simulink model "anjaneya_V5_2026-08-11"  (R2025a)
settings: Solver=VariableStepAuto  StartTime=0.0  StopTime=100  MaxStep=1e-3  RelTol=1e-6
settings Model: Creator=kuppa  LastModifiedBy=kuppa

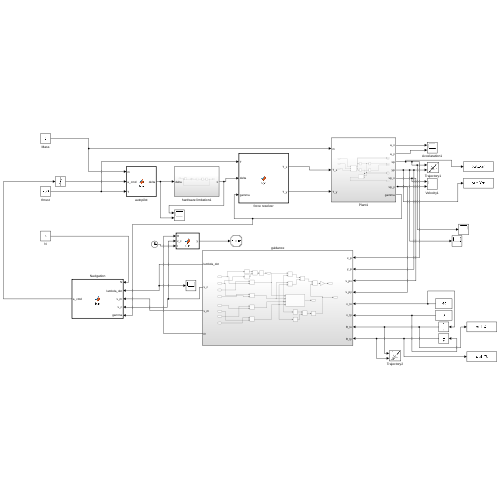
[thumbnail: Simulink's stored preview of the top-level diagram]
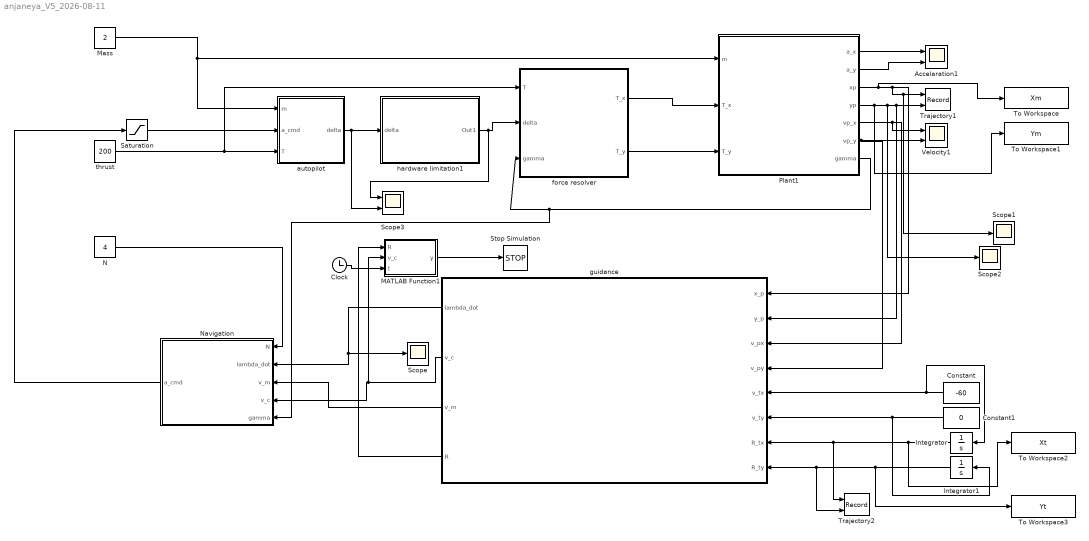
== system anjaneya_V5_2026-08-11 ==
  Accelaration1 : Scope  NumInputPorts=2
      settings: ActiveDisplayYMinimum=-670.09529615601855  ActiveDisplayYMaximum=430.47468331187889  DataLoggingVariableName=ScopeData2
  Clock : Clock
  Constant : Constant  Value=-60
  Constant1 : Constant  Value=0
  Integrator : Integrator  InitialCondition=3000
  Integrator1 : Integrator  InitialCondition=1500
  MATLAB Function1 : MATLAB Function  TreatAsAtomicUnit=on
  Mass : Constant  Value=2
  N : Constant  Value=4
  Navigation : MATLAB Function  TreatAsAtomicUnit=on
  Plant1 : Subsystem
  Saturation : Saturate  UpperLimit=108  LowerLimit=-108
  Scope : Scope
      settings: ActiveDisplayYMinimum=-0.71496170094090172  ActiveDisplayYMaximum=0.65598998004867615
  Scope1 : Scope
      settings: ActiveDisplayYMinimum=-25.430213641107127  ActiveDisplayYMaximum=35.257283778105105
  Scope2 : Scope
      settings: ActiveDisplayYMinimum=-57949.429144793568  ActiveDisplayYMaximum=306802.48338816618  DataLoggingVariableName=ScopeData4
  Scope3 : Scope  NumInputPorts=2
      settings: ActiveDisplayYMinimum=-0.11805254767904227  ActiveDisplayYMaximum=1.5944941621160178  DataLoggingVariableName=ScopeData5
  Stop Simulation : Stop
  To Workspace : ToWorkspace  VariableName=Xm  SaveFormat=Timeseries  SampleTime=-1
  To Workspace1 : ToWorkspace  VariableName=Ym  SaveFormat=Timeseries  SampleTime=-1
  To Workspace2 : ToWorkspace  VariableName=Xt  SaveFormat=Timeseries  SampleTime=-1
  To Workspace3 : ToWorkspace  VariableName=Yt  SaveFormat=Timeseries  SampleTime=-1
  Trajectory1 : Record  NumPorts=2.0  FileSettingsInternal="{\"entries\":[{\"content\":{\"excelSettings\":{\"content\":{},\"type\":\"Streamout.ExcelSettings\"},\"parquetSettings\":{\"content\":{},\"type\":\"Streamout.ParquetSettings\"}},\"type\":\"Streamout.FileSettingStorage\",\"uuid\":\"\"}],\"packageUris\":[\"http:\\/\\/schema.mathworks.com\\/mf0\\/streamout_blocks\\/R2020a\"],\"version\":\"1.0\"}"  FrameSettings=[0, 0]  Layout=[1 1]  SignalsInternal="{\"entries\":[{\"content\":{\"signals\":[{\"content\":{\"blockPath\":[],\"dimensions\":[1],\"domain\":\"\",\"lineColor\":\"#0072bd\",\"lineWidth\":2,\"port\":1,\"sid\":[\"\"],\"signalID\":1,\"signalName\":\"Plant1:3\"},\"type\":\"RecordBlkView.Signal\",\"uuid\":\"\"},{\"content\":{\"blockPath\":[],\"dimensions\":[1],\"domain\":\"\",\"lineColor\":\"#d95319\",\"lineWidth\":2,\"port\":2,\"sid\":[\"\"],\"signalID\":2,\"signalName\":\"Plant1:4\"},\"type\":\"RecordBlkView.Signal\",\"uuid\":\"\"}]},\"type\":\"RecordBlkView.InputSignals\",\"uuid\":\"\"}],\"packageUris\":[\"http:\\/\\/schema.mathworks.com\\/mf0\\/streamout_blocks\\/R2020a\"],\"version\":\"1.0\"}"  VisualizationBindings="{\"xyplotplugin\":{\"info\":[{\"series\":[],\"subplotID\":1}]}}"  CompatibilityTag=XY
  Trajectory2 : Record  NumPorts=2.0  FileSettingsInternal="{\"entries\":[{\"content\":{\"excelSettings\":{\"content\":{},\"type\":\"Streamout.ExcelSettings\"},\"parquetSettings\":{\"content\":{},\"type\":\"Streamout.ParquetSettings\"}},\"type\":\"Streamout.FileSettingStorage\",\"uuid\":\"\"}],\"packageUris\":[\"http:\\/\\/schema.mathworks.com\\/mf0\\/streamout_blocks\\/R2020a\"],\"version\":\"1.0\"}"  FrameSettings=[0, 0]  Layout=[1 1]  SignalsInternal="{\"entries\":[{\"content\":{\"signals\":[{\"content\":{\"blockPath\":[],\"dimensions\":[1],\"domain\":\"\",\"lineColor\":\"#edb120\",\"lineWidth\":2,\"port\":1,\"sid\":[\"\"],\"signalID\":1,\"signalName\":\"Integrator\"},\"type\":\"RecordBlkView.Signal\",\"uuid\":\"\"},{\"content\":{\"blockPath\":[],\"dimensions\":[1],\"domain\":\"\",\"lineColor\":\"#139fff\",\"plots\":[ 1 ],\"port\":2,\"sid\":[\"\"],\"signalID\":2,\"signalName\":\"Integrator1\"},\"type\":\"RecordBlkView.Signal\",\"uuid\":\"\"}]},\"type\":\"RecordBlkView.InputSignals\",\"uuid\":\"\"}],\"packageUris\":[\"http:\\/\\/schema.mathworks.com\\/mf0\\/streamout_blocks\\/R2020a\"],\"version\":\"1.0\"}"  VisualizationBindings="{\"xyplotplugin\":{\"info\":[{\"series\":[{\"bindingParametersList\":[{\"parameter\":\"Y-Axis\",\"signalID\":2,\"signalName\":\"Integrator1\"}],\"seriesID\":0}],\"subplotID\":1}]}}"  CompatibilityTag=XY
  Velocity1 : Scope  NumInputPorts=2
      settings: ActiveDisplayYMinimum=-149.61714228527322  ActiveDisplayYMaximum=359.76787547365052  DataLoggingVariableName=ScopeData3
  autopilot : MATLAB Function  TreatAsAtomicUnit=on
  force resolver : MATLAB Function  TreatAsAtomicUnit=on
  guidance : Subsystem
  hardware limitation1 : Subsystem
  thrust : Constant  Value=200
  wires:
  force resolver/1(T_x) -> Plant1/2(T_x)
  force resolver/2(T_y) -> Plant1/3(T_y)
  Plant1/7(gamma) -> Navigation/5(gamma), force resolver/3(gamma)
  Mass/1 -> autopilot/1(m), Plant1/1(m)
  thrust/1 -> autopilot/3(T), force resolver/1(T)
  Plant1/6(vp_y) -> guidance/4(v_py), Velocity1/2
  Plant1/5(vp_x) -> guidance/3(v_px), Velocity1/1
  Plant1/4(yp) -> To Workspace1/1, Scope2/1, guidance/2(y_p), Trajectory1/2
  Plant1/3(xp) -> To Workspace/1, guidance/1(x_p), Scope1/1, Trajectory1/1
  Plant1/2(a_y) -> Accelaration1/2
  Plant1/1(a_x) -> Accelaration1/1
  guidance/2(v_c) -> MATLAB Function1/2(v_c), Navigation/4(v_c)
  N/1 -> Navigation/1(N)
  Constant1/1 -> Integrator1/1, guidance/6(v_ty)
  Integrator/1 -> To Workspace2/1, Trajectory2/1, guidance/7(R_tx)
  Integrator1/1 -> Trajectory2/2, guidance/8(R_ty), To Workspace3/1
  Navigation/1(a_cmd) -> Saturation/1
  MATLAB Function1/1(y) -> Stop Simulation/1
  Clock/1 -> MATLAB Function1/3(t)
  Constant/1 -> guidance/5(v_tx), Integrator/1
  guidance/3(v_m) -> Navigation/3(v_m)
  Saturation/1 -> autopilot/2(a_cmd)
  guidance/1(lambda_dot) -> Navigation/2(lambda_dot), Scope/1
  guidance/4(R) -> MATLAB Function1/1(R)
  autopilot/1(delta) -> Scope3/2, hardware limitation1/1(delta)
  hardware limitation1/1(Out1) -> Scope3/1, force resolver/2(delta)

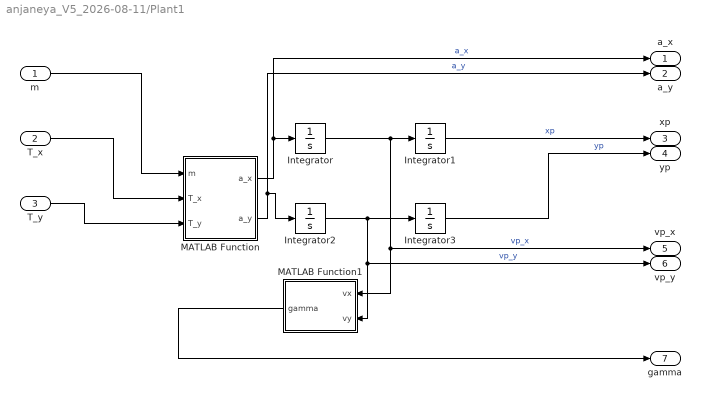
== system anjaneya_V5_2026-08-11/Plant1 ==
  m : Inport
  T_x : Inport  Port=2
  T_y : Inport  Port=3
  Integrator : Integrator  InitialCondition=230
  Integrator1 : Integrator
  Integrator2 : Integrator  InitialCondition=30
  Integrator3 : Integrator
  MATLAB Function : MATLAB Function  TreatAsAtomicUnit=on
  MATLAB Function1 : MATLAB Function  TreatAsAtomicUnit=on
  a_x : Outport
  a_y : Outport  Port=2
  xp : Outport  Port=3
  yp : Outport  Port=4
  vp_x : Outport  Port=5
  vp_y : Outport  Port=6
  gamma : Outport  Port=7
  wires:
  m/1 -> MATLAB Function/1(m)
  MATLAB Function/2(a_y) -> Integrator2/1, a_y/1  "a_y"
  Integrator/1 -> Integrator1/1, vp_x/1, MATLAB Function1/1(vx)  "vp_x"
  Integrator2/1 -> Integrator3/1, vp_y/1, MATLAB Function1/2(vy)  "vp_y"
  T_x/1 -> MATLAB Function/2(T_x)
  T_y/1 -> MATLAB Function/3(T_y)
  MATLAB Function/1(a_x) -> Integrator/1, a_x/1  "a_x"
  Integrator3/1 -> yp/1  "yp"
  Integrator1/1 -> xp/1  "xp"
  MATLAB Function1/1(gamma) -> gamma/1

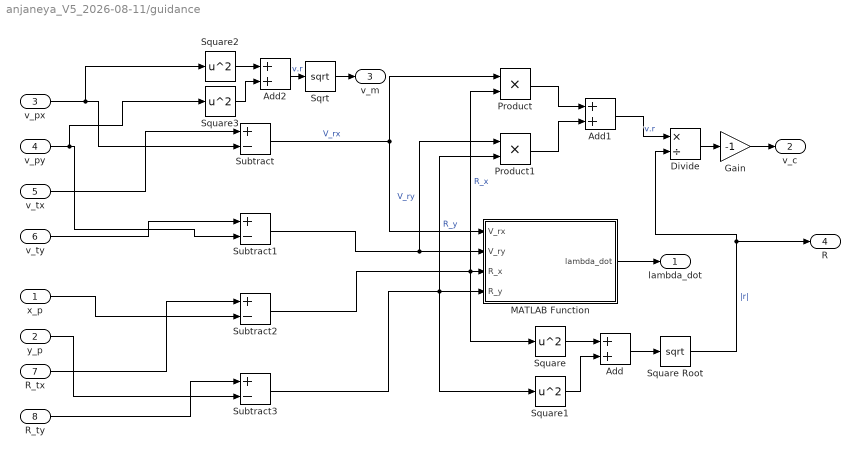
== system anjaneya_V5_2026-08-11/guidance ==
  x_p : Inport
  y_p : Inport  Port=2
  v_px : Inport  Port=3
  v_py : Inport  Port=4
  v_tx : Inport  Port=5
  v_ty : Inport  Port=6
  R_tx : Inport  Port=7
  R_ty : Inport  Port=8
  Add : Sum
  Add1 : Sum
  Add2 : Sum
  Divide : Product  Inputs=*/
  Gain : Gain  Gain=-1
  MATLAB Function : MATLAB Function  TreatAsAtomicUnit=on
  Product : Product
  Product1 : Product
  Sqrt : Sqrt
  Square{,1..3} (4 alike) : Math  Operator=square
  Square Root : Sqrt
  Subtract{,1..3} (4 alike) : Sum  Inputs=+-
  lambda_dot : Outport
  v_c : Outport  Port=2
  v_m : Outport  Port=3
  R : Outport  Port=4
  wires:
  x_p/1 -> Subtract2/2
  v_tx/1 -> Subtract/1
  v_px/1 -> Square2/1, Subtract/2
  Subtract/1 -> Product/1, MATLAB Function/1(V_rx)  "V_rx"
  v_ty/1 -> Subtract1/1
  v_py/1 -> Square3/1, Subtract1/2
  Subtract1/1 -> MATLAB Function/2(V_ry), Product1/1  "V_ry"
  R_tx/1 -> Subtract2/1
  R_ty/1 -> Subtract3/1
  y_p/1 -> Subtract3/2
  Subtract2/1 -> Square/1, MATLAB Function/3(R_x), Product/2  "R_x"
  Subtract3/1 -> MATLAB Function/4(R_y), Product1/2, Square1/1  "R_y"
  MATLAB Function/1(lambda_dot) -> lambda_dot/1
  Square/1 -> Add/1
  Square1/1 -> Add/2
  Add/1 -> Square Root/1
  Square Root/1 -> Divide/2, R/1  "|r|"
  Product/1 -> Add1/1
  Product1/1 -> Add1/2
  Add1/1 -> Divide/1  "v.r"
  Divide/1 -> Gain/1
  Gain/1 -> v_c/1
  Square2/1 -> Add2/1
  Square3/1 -> Add2/2
  Add2/1 -> Sqrt/1  "v.r"
  Sqrt/1 -> v_m/1

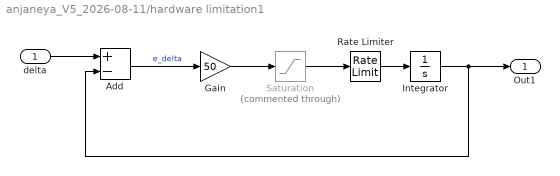
== system anjaneya_V5_2026-08-11/hardware limitation1 ==
  delta : Inport
  Add : Sum  Inputs=+-
  Gain : Gain  Gain=50
  Integrator : Integrator  LimitOutput=on  UpperSaturationLimit=0.26  LowerSaturationLimit=-0.26
  Rate Limiter : RateLimiter  RisingSlewLimit=3  FallingSlewLimit=-3  SampleTimeMode=inherited
  Saturation : Saturate  Commented=through  UpperLimit=0.052  LowerLimit=-0.052
  Out1 : Outport
  wires:
  Rate Limiter/1 -> Integrator/1
  Add/1 -> Gain/1  "e_delta"
  delta/1 -> Add/1
  Saturation/1 -> Rate Limiter/1
  Gain/1 -> Saturation/1
  Integrator/1 -> Add/2, Out1/1

== matlab function anjaneya_V5_2026-08-11/Navigation ==
  data: N input; a_cmd output; lambda_dot input; v_m input; v_c input; gamma input
function a_cmd = fcn(N, lambda_dot, v_m, v_c, gamma)
    g = 9.81;

    if v_c > 0 
        a_guide = N * v_m * lambda_dot;
    else
        a_guide = 0;
    end
    
    a_grav = g * cos(gamma);

    a_cmd = a_guide + a_grav;
end

== matlab function anjaneya_V5_2026-08-11/guidance/MATLAB Function ==
  data: V_rx input; lambda_dot output; V_ry input; R_x input; R_y input
function lambda_dot = fcn(V_rx, V_ry, R_x, R_y)

R_square = R_x*R_x + R_y*R_y;
lambda_dot = (R_x*V_ry - R_y*V_rx )/R_square ;

== matlab function anjaneya_V5_2026-08-11/MATLAB Function1 ==
  data: R input; v_c input; y output; t input
function y = fcn(R, v_c, t)
    if t > 0.05 && (R < 0.5 || v_c <= 0)
        y = 1;
    else
        y = 0;
    end
end

== matlab function anjaneya_V5_2026-08-11/Plant1/MATLAB Function ==
  data: m input; T_x input; T_y input; a_x output; a_y output
function [a_x,a_y]= fcn(m, T_x, T_y)

g = 9.81;
a_x = (T_x)/m;
a_y = ((T_y)/m -g);

== matlab function anjaneya_V5_2026-08-11/Plant1/MATLAB Function1 ==
  data: vx input; gamma output; vy input
function gamma = fcn(vx, vy)

gamma = atan2(vy,vx);

== matlab function anjaneya_V5_2026-08-11/force resolver ==
  data: T input; delta input; gamma input; T_x output; T_y output
function [T_x , T_y] = fcn(T , delta , gamma)

theta_T = delta + gamma;
T_x = T*cos(theta_T);
T_y = T*sin(theta_T);

== matlab function anjaneya_V5_2026-08-11/autopilot ==
  data: m input; a_cmd input; delta output; T input
function delta = fcn(m, a_cmd, T)
    s = m * a_cmd / T;
    s = max(min(s, 0.99), -0.99);
    delta = asin(s);
end
